simulink model "tb_mcu_closed_loop"  (R2026b)
values from neighbouring files (symbols this model uses):
  P = evalin('base', 'P')    [elec_harness.m]    (also in mcu_can1_roundtrip.m; mcu_can2_roundtrip.m; mcu_cl_input.m; mcu_ctrl_harness.m)
  Ts = prm(1)    [mcu_cl_track_dyn.m]    (also in mcu_ctrl_harness.m = evalin('base', tsExpr))
undefined symbols (not defined in the file or in its folder): DiscIntNeverNeededParam
libraries: simulink x57, robotmobilelib x1
(part 1 of 2)
settings Model: Creator=aomar  LastModifiedBy=aomar

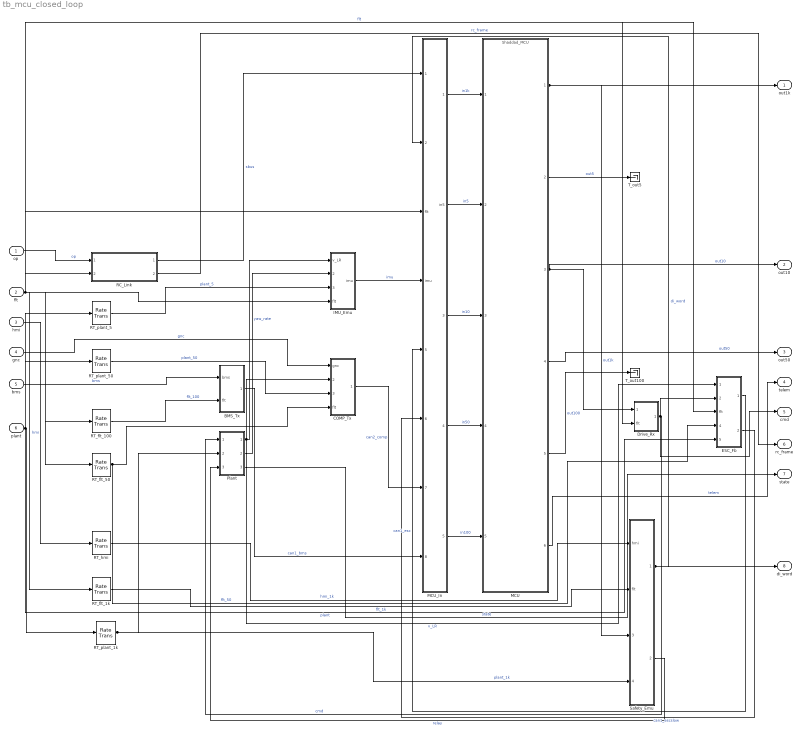
== system tb_mcu_closed_loop ==
  op : Inport  OutDataTypeStr=Bus: Bus_OperatorCmd  SampleTime=Ts.ctrl  BusOutputAsStruct=on
  flt : Inport  Port=2  OutDataTypeStr=Bus: Bus_FaultInject  SampleTime=Ts.ctrl  BusOutputAsStruct=on
  hmi : Inport  Port=3  OutDataTypeStr=Bus: Bus_HmiInputs  SampleTime=Ts.ctrl  BusOutputAsStruct=on
  gnc : Inport  Port=4  OutDataTypeStr=Bus: Bus_GncCmd  SampleTime=Ts.comm  BusOutputAsStruct=on
  bms : Inport  Port=5  OutDataTypeStr=Bus: Bus_BMS_Telemetry  SampleTime=Ts.hk  BusOutputAsStruct=on
  plant : Inport  Port=6  OutDataTypeStr=double  PortDimensions=9  SampleTime=Ts.ctrl
  BMS_Tx : Subsystem
  COMP_Tx : Subsystem
  Drive_Rx : Subsystem
  ESC_Fb : Subsystem
  IMU_Emu : Subsystem
  MCU : ModelReference  ModelNameDialog=Shaddad_MCU  SimulationMode=Normal  ModelReferenceVersion=1.1
  MCU_In : Subsystem
  Plant : Subsystem
  RC_Link : Subsystem  ReferencedSubsystem=RC_Link_Sim
  RT_flt_100 : RateTransition  InitialCondition=P.ic.Bus_FaultInject  OutPortSampleTime=Ts.hk
  RT_flt_1k : RateTransition  InitialCondition=P.ic.Bus_FaultInject  OutPortSampleTime=Ts.base
  RT_flt_50 : RateTransition  InitialCondition=P.ic.Bus_FaultInject  OutPortSampleTime=Ts.comm
  RT_hmi : RateTransition  InitialCondition=P.ic.Bus_HmiInputs  OutPortSampleTime=Ts.base
  RT_plant_1k : RateTransition  InitialCondition=[1 0 0 0 0 0 0 0 0]  OutPortSampleTime=Ts.base
  RT_plant_5 : RateTransition  InitialCondition=[1 0 0 0 0 0 0 0 0]  OutPortSampleTime=Ts.imu
  RT_plant_50 : RateTransition  InitialCondition=[1 0 0 0 0 0 0 0 0]  OutPortSampleTime=Ts.comm
  Safety_Emu : Subsystem
  T_out100 : Terminator
  T_out5 : Terminator
  out1k : Outport  OutDataTypeStr=Bus: Bus_McuOut1k
  out10 : Outport  Port=2  OutDataTypeStr=Bus: Bus_McuOut10
  out50 : Outport  Port=3  OutDataTypeStr=Bus: Bus_McuOut50
  telem : Outport  Port=4  OutDataTypeStr=Bus: Bus_FwTelemetry
  cmd : Outport  Port=5  OutDataTypeStr=Bus: Bus_DriveCmd
  rc_frame : Outport  Port=6  OutDataTypeStr=Bus: Bus_RcFrame
  state : Outport  Port=7  OutDataTypeStr=double
  di_word : Outport  Port=8  OutDataTypeStr=uint16
  wires:
  op/1 -> RC_Link/1  "op"
  hmi/1 -> RT_hmi/1  "hmi"
  gnc/1 -> COMP_Tx/1(gnc)  "gnc"
  bms/1 -> BMS_Tx/1(bms)  "bms"
  RT_plant_5/1 -> IMU_Emu/3(plant)  "plant_5"
  RT_plant_50/1 -> COMP_Tx/3(plant)  "plant_50"
  RT_flt_100/1 -> BMS_Tx/2(flt)  "flt_100"
  RT_flt_50/1 -> COMP_Tx/4(flt), ESC_Fb/4(flt_50)  "flt_50"
  RT_hmi/1 -> Safety_Emu/1(hmi)  "hmi_1k"
  RT_flt_1k/1 -> Safety_Emu/2(flt)  "flt_1k"
  RT_plant_1k/1 -> Plant/2(plant), Safety_Emu/4(plant)  "plant_1k"
  RC_Link/1 -> MCU_In/1(sbus)  "sbus"
  RC_Link/2 -> rc_frame/1  "rc_frame"
  BMS_Tx/1(frames) -> MCU_In/8(can1_bms)  "can1_bms"
  Plant/1(v_LR) -> IMU_Emu/1(v_LR), COMP_Tx/2(v_LR), ESC_Fb/1(v_LR)  "v_LR"
  Plant/2(yaw_rate) -> IMU_Emu/2(yaw_rate)  "yaw_rate"
  Plant/3(state) -> state/1  "state"
  IMU_Emu/1(imu) -> MCU_In/4(imu)  "imu"
  COMP_Tx/1(frame) -> MCU_In/7(can2_comp)  "can2_comp"
  MCU_In/1(in1k) -> MCU/1  "in1k"
  MCU_In/2(in5) -> MCU/2  "in5"
  MCU_In/3(in10) -> MCU/3  "in10"
  MCU_In/4(in50) -> MCU/4  "in50"
  MCU_In/5(in100) -> MCU/5  "in100"
  MCU/1 -> Safety_Emu/3(out1k), out1k/1  "out1k"
  MCU/2 -> T_out5/1  "out5"
  MCU/3 -> Drive_Rx/1(out10), out10/1  "out10"
  MCU/4 -> out50/1  "out50"
  MCU/5 -> T_out100/1  "out100"
  MCU/6 -> telem/1  "telem"
  Safety_Emu/1(di_word) -> MCU_In/2(di_word), di_word/1  "di_word"
  Safety_Emu/2(relay) -> Plant/3(relay)  "relay"
  Drive_Rx/1(cmd) -> Plant/1(cmd), ESC_Fb/2(cmd), cmd/1  "cmd"
  ESC_Fb/1(esc_fast) -> MCU_In/5(can1_esc)  "can1_esc"
  ESC_Fb/2(esc_slow) -> MCU_In/6(can1_escslow)  "can1_escslow"
  flt/1 -> RT_flt_1k/1, RT_flt_50/1, Drive_Rx/2(flt), RT_flt_100/1, ESC_Fb/3(flt), MCU_In/3(flt), RC_Link/2, IMU_Emu/4(flt)  "flt"
  plant/1 -> RT_plant_1k/1, RT_plant_5/1, RT_plant_50/1, ESC_Fb/5(plant)  "plant"

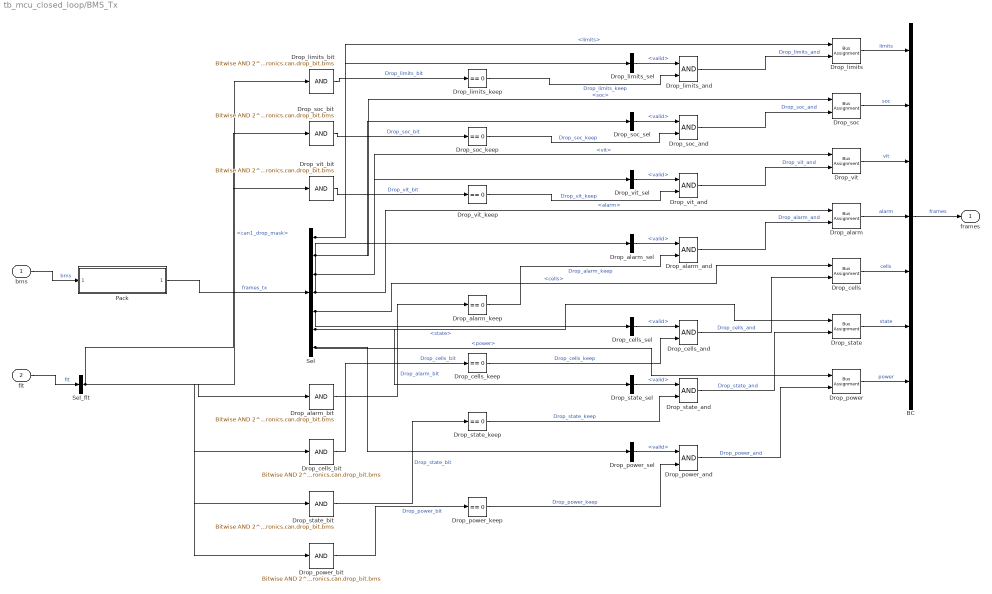
== system tb_mcu_closed_loop/BMS_Tx ==
  bms : Inport
  flt : Inport  Port=2
  BC : BusCreator  Inputs=7  OutDataTypeStr=Bus: Bus_Can1_Bms  NonVirtualBus=on
      settings: InheritFromInputs=off
  Drop_alarm : BusAssignment  AssignedSignals=valid
  Drop_alarm_and : Logic  AllPortsSameDT=off  OutDataTypeStr=boolean
  Drop_alarm_bit : simulink/Logic and Bit Operations/Bitwise Operator  logicop=AND  UseBitMask=on  BitMask=2^P.electronics.can.drop_bit.bms  BitMaskRealWorld=Stored Integer
  Drop_alarm_keep : simulink/Logic and Bit Operations/Compare To Zero  relop===  OutDataTypeStr=boolean
  Drop_alarm_sel : BusSelector  OutputSignals=valid
  Drop_cells : BusAssignment  AssignedSignals=valid
  Drop_cells_and : Logic  AllPortsSameDT=off  OutDataTypeStr=boolean
  Drop_cells_bit : simulink/Logic and Bit Operations/Bitwise Operator  logicop=AND  UseBitMask=on  BitMask=2^P.electronics.can.drop_bit.bms  BitMaskRealWorld=Stored Integer
  Drop_cells_keep : simulink/Logic and Bit Operations/Compare To Zero  relop===  OutDataTypeStr=boolean
  Drop_cells_sel : BusSelector  OutputSignals=valid
  Drop_limits : BusAssignment  AssignedSignals=valid
  Drop_limits_and : Logic  AllPortsSameDT=off  OutDataTypeStr=boolean
  Drop_limits_bit : simulink/Logic and Bit Operations/Bitwise Operator  logicop=AND  UseBitMask=on  BitMask=2^P.electronics.can.drop_bit.bms  BitMaskRealWorld=Stored Integer
  Drop_limits_keep : simulink/Logic and Bit Operations/Compare To Zero  relop===  OutDataTypeStr=boolean
  Drop_limits_sel : BusSelector  OutputSignals=valid
  Drop_power : BusAssignment  AssignedSignals=valid
  Drop_power_and : Logic  AllPortsSameDT=off  OutDataTypeStr=boolean
  Drop_power_bit : simulink/Logic and Bit Operations/Bitwise Operator  logicop=AND  UseBitMask=on  BitMask=2^P.electronics.can.drop_bit.bms  BitMaskRealWorld=Stored Integer
  Drop_power_keep : simulink/Logic and Bit Operations/Compare To Zero  relop===  OutDataTypeStr=boolean
  Drop_power_sel : BusSelector  OutputSignals=valid
  Drop_soc : BusAssignment  AssignedSignals=valid
  Drop_soc_and : Logic  AllPortsSameDT=off  OutDataTypeStr=boolean
  Drop_soc_bit : simulink/Logic and Bit Operations/Bitwise Operator  logicop=AND  UseBitMask=on  BitMask=2^P.electronics.can.drop_bit.bms  BitMaskRealWorld=Stored Integer
  Drop_soc_keep : simulink/Logic and Bit Operations/Compare To Zero  relop===  OutDataTypeStr=boolean
  Drop_soc_sel : BusSelector  OutputSignals=valid
  Drop_state : BusAssignment  AssignedSignals=valid
  Drop_state_and : Logic  AllPortsSameDT=off  OutDataTypeStr=boolean
  Drop_state_bit : simulink/Logic and Bit Operations/Bitwise Operator  logicop=AND  UseBitMask=on  BitMask=2^P.electronics.can.drop_bit.bms  BitMaskRealWorld=Stored Integer
  Drop_state_keep : simulink/Logic and Bit Operations/Compare To Zero  relop===  OutDataTypeStr=boolean
  Drop_state_sel : BusSelector  OutputSignals=valid
  Drop_vit : BusAssignment  AssignedSignals=valid
  Drop_vit_and : Logic  AllPortsSameDT=off  OutDataTypeStr=boolean
  Drop_vit_bit : simulink/Logic and Bit Operations/Bitwise Operator  logicop=AND  UseBitMask=on  BitMask=2^P.electronics.can.drop_bit.bms  BitMaskRealWorld=Stored Integer
  Drop_vit_keep : simulink/Logic and Bit Operations/Compare To Zero  relop===  OutDataTypeStr=boolean
  Drop_vit_sel : BusSelector  OutputSignals=valid
  Pack : Subsystem  ReferencedSubsystem=bms_can_pack
  Sel : BusSelector  OutputSignals=limits,soc,vit,alarm,cells,state,power
  Sel_flt : BusSelector  OutputSignals=can1_drop_mask
  frames : Outport
  wires:
  bms/1 -> Pack/1  "bms"
  flt/1 -> Sel_flt/1  "flt"
  Sel_flt/1 -> Drop_limits_bit/1, Drop_soc_bit/1, Drop_vit_bit/1, Drop_power_bit/1, Drop_state_bit/1, Drop_cells_bit/1, Drop_alarm_bit/1  "<can1_drop_mask>"
  Pack/1 -> Sel/1  "frames_tx"
  Sel/1 -> Drop_limits/1, Drop_limits_sel/1  "<limits>"
  Sel/2 -> Drop_soc/1, Drop_soc_sel/1  "<soc>"
  Sel/3 -> Drop_vit/1, Drop_vit_sel/1  "<vit>"
  Sel/4 -> Drop_alarm/1, Drop_alarm_sel/1  "<alarm>"
  Sel/5 -> Drop_cells/1, Drop_cells_sel/1  "<cells>"
  Sel/6 -> Drop_state_sel/1, Drop_state/1  "<state>"
  Sel/7 -> Drop_power_sel/1, Drop_power/1  "<power>"
  Drop_limits_bit/1 -> Drop_limits_keep/1  "Drop_limits_bit"
  Drop_soc_bit/1 -> Drop_soc_keep/1  "Drop_soc_bit"
  Drop_vit_bit/1 -> Drop_vit_keep/1  "Drop_vit_bit"
  Drop_alarm_bit/1 -> Drop_alarm_keep/1  "Drop_alarm_bit"
  Drop_cells_bit/1 -> Drop_cells_keep/1  "Drop_cells_bit"
  Drop_state_bit/1 -> Drop_state_keep/1  "Drop_state_bit"
  Drop_power_bit/1 -> Drop_power_keep/1  "Drop_power_bit"
  Drop_limits_keep/1 -> Drop_limits_and/2  "Drop_limits_keep"
  Drop_soc_keep/1 -> Drop_soc_and/2  "Drop_soc_keep"
  Drop_vit_keep/1 -> Drop_vit_and/2  "Drop_vit_keep"
  Drop_alarm_keep/1 -> Drop_alarm_and/2  "Drop_alarm_keep"
  Drop_cells_keep/1 -> Drop_cells_and/2  "Drop_cells_keep"
  Drop_state_keep/1 -> Drop_state_and/2  "Drop_state_keep"
  Drop_power_keep/1 -> Drop_power_and/2  "Drop_power_keep"
  Drop_limits_sel/1 -> Drop_limits_and/1  "<valid>"
  Drop_soc_sel/1 -> Drop_soc_and/1  "<valid>"
  Drop_vit_sel/1 -> Drop_vit_and/1  "<valid>"
  Drop_alarm_sel/1 -> Drop_alarm_and/1  "<valid>"
  Drop_cells_sel/1 -> Drop_cells_and/1  "<valid>"
  Drop_state_sel/1 -> Drop_state_and/1  "<valid>"
  Drop_power_sel/1 -> Drop_power_and/1  "<valid>"
  Drop_limits_and/1 -> Drop_limits/2  "Drop_limits_and"
  Drop_soc_and/1 -> Drop_soc/2  "Drop_soc_and"
  Drop_vit_and/1 -> Drop_vit/2  "Drop_vit_and"
  Drop_alarm_and/1 -> Drop_alarm/2  "Drop_alarm_and"
  Drop_cells_and/1 -> Drop_cells/2  "Drop_cells_and"
  Drop_state_and/1 -> Drop_state/2  "Drop_state_and"
  Drop_power_and/1 -> Drop_power/2  "Drop_power_and"
  Drop_limits/1 -> BC/1  "limits"
  Drop_soc/1 -> BC/2  "soc"
  Drop_vit/1 -> BC/3  "vit"
  Drop_alarm/1 -> BC/4  "alarm"
  Drop_cells/1 -> BC/5  "cells"
  Drop_state/1 -> BC/6  "state"
  Drop_power/1 -> BC/7  "power"
  BC/1 -> frames/1  "frames"

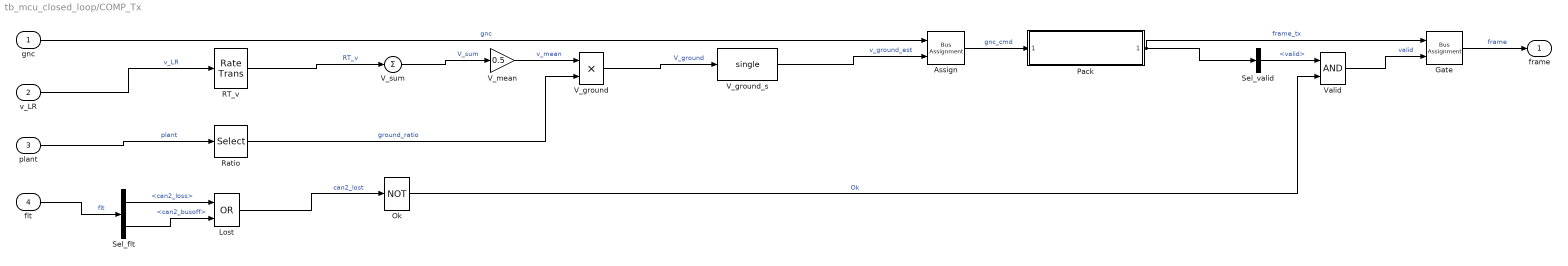
== system tb_mcu_closed_loop/COMP_Tx ==
  gnc : Inport
  v_LR : Inport  Port=2
  plant : Inport  Port=3
  flt : Inport  Port=4
  Assign : BusAssignment  AssignedSignals=v_ground_est
  Gate : BusAssignment  AssignedSignals=valid
  Lost : Logic  Operator=OR  AllPortsSameDT=off  OutDataTypeStr=boolean
  Ok : Logic  Operator=NOT  Inputs=1  AllPortsSameDT=off  OutDataTypeStr=boolean
  Pack : Subsystem  ReferencedSubsystem=can2_comp_cmd_pack
  RT_v : RateTransition  InitialCondition=[0 0]  OutPortSampleTime=Ts.comm
  Ratio : Selector  InputPortWidth=9  IndexOptions=Index vector (dialog)  Indices=4  OutputSizes=1
  Sel_flt : BusSelector  OutputSignals=can2_loss,can2_busoff
  Sel_valid : BusSelector  OutputSignals=valid
  V_ground : Product  Inputs=**
  V_ground_s : DataTypeConversion  OutDataTypeStr=single  RndMeth=Round
  V_mean : Gain  Gain=0.5
  V_sum : Sum  Inputs=+
  Valid : Logic  AllPortsSameDT=off  OutDataTypeStr=boolean
  frame : Outport
  wires:
  gnc/1 -> Assign/1  "gnc"
  v_LR/1 -> RT_v/1  "v_LR"
  plant/1 -> Ratio/1  "plant"
  flt/1 -> Sel_flt/1  "flt"
  Sel_flt/1 -> Lost/1  "<can2_loss>"
  Sel_flt/2 -> Lost/2  "<can2_busoff>"
  Lost/1 -> Ok/1  "can2_lost"
  RT_v/1 -> V_sum/1  "RT_v"
  Ratio/1 -> V_ground/2  "ground_ratio"
  V_sum/1 -> V_mean/1  "V_sum"
  Ok/1 -> Valid/2  "Ok"
  V_mean/1 -> V_ground/1  "v_mean"
  V_ground/1 -> V_ground_s/1  "V_ground"
  V_ground_s/1 -> Assign/2  "v_ground_est"
  Assign/1 -> Pack/1  "gnc_cmd"
  Pack/1 -> Sel_valid/1, Gate/1  "frame_tx"
  Sel_valid/1 -> Valid/1  "<valid>"
  Valid/1 -> Gate/2  "valid"
  Gate/1 -> frame/1  "frame"

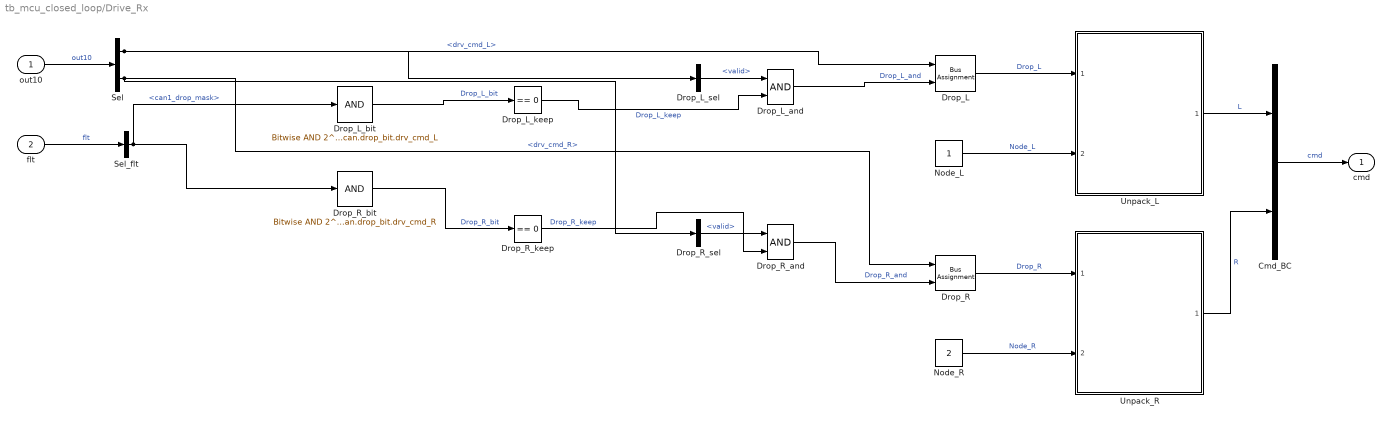
== system tb_mcu_closed_loop/Drive_Rx ==
  out10 : Inport
  flt : Inport  Port=2
  Cmd_BC : BusCreator  Inputs=2  OutDataTypeStr=Bus: Bus_DriveCmd  NonVirtualBus=on
      settings: InheritFromInputs=off
  Drop_L : BusAssignment  AssignedSignals=valid
  Drop_L_and : Logic  AllPortsSameDT=off  OutDataTypeStr=boolean
  Drop_L_bit : simulink/Logic and Bit Operations/Bitwise Operator  logicop=AND  UseBitMask=on  BitMask=2^P.electronics.can.drop_bit.drv_cmd_L  BitMaskRealWorld=Stored Integer
  Drop_L_keep : simulink/Logic and Bit Operations/Compare To Zero  relop===  OutDataTypeStr=boolean
  Drop_L_sel : BusSelector  OutputSignals=valid
  Drop_R : BusAssignment  AssignedSignals=valid
  Drop_R_and : Logic  AllPortsSameDT=off  OutDataTypeStr=boolean
  Drop_R_bit : simulink/Logic and Bit Operations/Bitwise Operator  logicop=AND  UseBitMask=on  BitMask=2^P.electronics.can.drop_bit.drv_cmd_R  BitMaskRealWorld=Stored Integer
  Drop_R_keep : simulink/Logic and Bit Operations/Compare To Zero  relop===  OutDataTypeStr=boolean
  Drop_R_sel : BusSelector  OutputSignals=valid
  Node_L : Constant  OutDataTypeStr=uint8  SampleTime=Ts.ctrl
  Node_R : Constant  Value=2  OutDataTypeStr=uint8  SampleTime=Ts.ctrl
  Sel : BusSelector  OutputSignals=can1_drv.drv_cmd_L,can1_drv.drv_cmd_R
  Sel_flt : BusSelector  OutputSignals=can1_drop_mask
  Unpack_L : Subsystem  ReferencedSubsystem=drive_cmd_unpack
  Unpack_R : Subsystem  ReferencedSubsystem=drive_cmd_unpack
  cmd : Outport
  wires:
  out10/1 -> Sel/1  "out10"
  flt/1 -> Sel_flt/1  "flt"
  Sel/1 -> Drop_L_sel/1, Drop_L/1  "<drv_cmd_L>"
  Sel/2 -> Drop_R/1, Drop_R_sel/1  "<drv_cmd_R>"
  Sel_flt/1 -> Drop_R_bit/1, Drop_L_bit/1  "<can1_drop_mask>"
  Drop_L_bit/1 -> Drop_L_keep/1  "Drop_L_bit"
  Drop_R_bit/1 -> Drop_R_keep/1  "Drop_R_bit"
  Drop_L_keep/1 -> Drop_L_and/2  "Drop_L_keep"
  Drop_R_keep/1 -> Drop_R_and/2  "Drop_R_keep"
  Drop_L_sel/1 -> Drop_L_and/1  "<valid>"
  Drop_R_sel/1 -> Drop_R_and/1  "<valid>"
  Drop_L_and/1 -> Drop_L/2  "Drop_L_and"
  Drop_R_and/1 -> Drop_R/2  "Drop_R_and"
  Node_L/1 -> Unpack_L/2  "Node_L"
  Node_R/1 -> Unpack_R/2  "Node_R"
  Drop_L/1 -> Unpack_L/1  "Drop_L"
  Drop_R/1 -> Unpack_R/1  "Drop_R"
  Unpack_L/1 -> Cmd_BC/1  "L"
  Unpack_R/1 -> Cmd_BC/2  "R"
  Cmd_BC/1 -> cmd/1  "cmd"

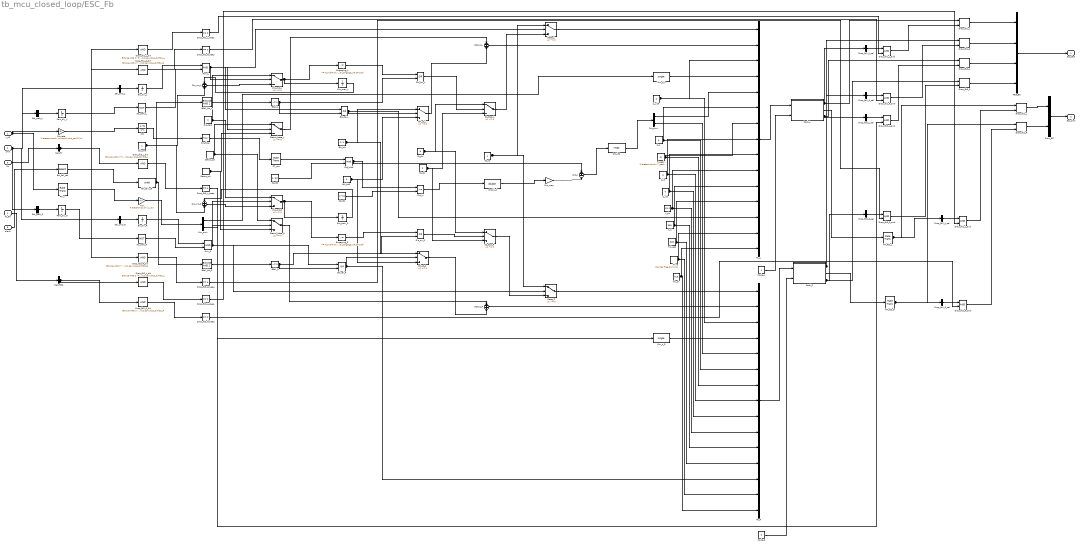
== system tb_mcu_closed_loop/ESC_Fb ==
  v_LR : Inport
  cmd : Inport  Port=2
  flt : Inport  Port=3
  flt_50 : Inport  Port=4
  plant : Inport  Port=5
  Alive : simulink/Sources/Counter Free-Running  NumBits=8  tsamp=Ts.ctrl
  Bfail_L : simulink/Logic and Bit Operations/Compare To Zero  relop=~=  OutDataTypeStr=boolean
  Bfail_R : simulink/Logic and Bit Operations/Compare To Zero  relop=~=  OutDataTypeStr=boolean
  Bfail_bit_L : simulink/Logic and Bit Operations/Bitwise Operator  logicop=AND  UseBitMask=on  BitMask=1  BitMaskRealWorld=Stored Integer
  Bfail_bit_R : simulink/Logic and Bit Operations/Bitwise Operator  logicop=AND  UseBitMask=on  BitMask=2  BitMaskRealWorld=Stored Integer
  Brk_bit : Constant  Value=2^4  OutDataTypeStr=uint16  SampleTime=Ts.ctrl
  Brk_bit0 : Constant  Value=0  OutDataTypeStr=uint16  SampleTime=Ts.ctrl
  Brk_fail_sel : Selector  InputPortWidth=9  IndexOptions=Index vector (dialog)  Indices=6  OutputSizes=1
  Brk_fail_u8 : DataTypeConversion  OutDataTypeStr=uint8  RndMeth=Round
  Brk_rel_L : Logic  Operator=OR  AllPortsSameDT=off  OutDataTypeStr=boolean
  Brk_rel_R : Logic  Operator=OR  AllPortsSameDT=off  OutDataTypeStr=boolean
  Brk_st_L : Switch  Criteria=u2 ~= 0  SaturateOnIntegerOverflow=off  InputSameDT=off
  Brk_st_R : Switch  Criteria=u2 ~= 0  SaturateOnIntegerOverflow=off  InputSameDT=off
  C2p31 : Constant  Value=2^31  OutDataTypeStr=double  SampleTime=Ts.ctrl
  C2p32 : Constant  Value=2^32  OutDataTypeStr=double  SampleTime=Ts.ctrl
  Cnt : DiscreteIntegrator  InitialCondition=[0 0]  SampleTime=Ts.base  ICPrevOutput=DiscIntNeverNeededParam  ICPrevScaledInput=DiscIntNeverNeededParam
  Cnt_dmx : Demux  Outputs=2
  Cnt_floor : Rounding
  Cnt_hi : RelationalOperator  OutDataTypeStr=boolean  RndMeth=Simplest  InputSameDT=off
  Cnt_hi_d : DataTypeConversion  OutDataTypeStr=double  RndMeth=Round
  Cnt_i32 : DataTypeConversion  OutDataTypeStr=int32  RndMeth=Round
  Cnt_mod : Math  Operator=mod
  Cnt_rate : Gain  Gain=P.electronics.drv.k_v2w*P.electronics.drv.enc_cpr/(2*pi)
  Cnt_s : Sum  Inputs=+-
  Cnt_wrap : Gain  Gain=2^32
  Dis_cnt_L : Switch  Criteria=u2 ~= 0  SaturateOnIntegerOverflow=off  InputSameDT=off
  Dis_cnt_R : Switch  Criteria=u2 ~= 0  SaturateOnIntegerOverflow=off  InputSameDT=off
  Dis_inc_L : Sum  OutDataTypeStr=uint16  SaturateOnIntegerOverflow=on
  Dis_inc_R : Sum  OutDataTypeStr=uint16  SaturateOnIntegerOverflow=on
  Dis_on_L : Logic  Operator=OR  AllPortsSameDT=off  OutDataTypeStr=boolean
  Dis_on_R : Logic  Operator=OR  AllPortsSameDT=off  OutDataTypeStr=boolean
  Dis_one : Constant  OutDataTypeStr=uint16  SampleTime=Ts.ctrl
  Dis_prev_L : UnitDelay  InitialCondition=1000  SampleTime=Ts.ctrl
  Dis_prev_R : UnitDelay  InitialCondition=1000  SampleTime=Ts.ctrl
  Dis_zero : Constant  Value=0  OutDataTypeStr=uint16  SampleTime=Ts.ctrl
  Drop_fb1_L : BusAssignment  AssignedSignals=valid
  Drop_fb1_L_and : Logic  AllPortsSameDT=off  OutDataTypeStr=boolean
  Drop_fb1_L_bit : simulink/Logic and Bit Operations/Bitwise Operator  logicop=AND  UseBitMask=on  BitMask=2^P.electronics.can.drop_bit.fb1_L  BitMaskRealWorld=Stored Integer
  Drop_fb1_L_keep : simulink/Logic and Bit Operations/Compare To Zero  relop===  OutDataTypeStr=boolean
  Drop_fb1_L_sel : BusSelector  OutputSignals=valid
  Drop_fb1_R : BusAssignment  AssignedSignals=valid
  Drop_fb1_R_and : Logic  AllPortsSameDT=off  OutDataTypeStr=boolean
  Drop_fb1_R_bit : simulink/Logic and Bit Operations/Bitwise Operator  logicop=AND  UseBitMask=on  BitMask=2^P.electronics.can.drop_bit.fb1_R  BitMaskRealWorld=Stored Integer
  Drop_fb1_R_keep : simulink/Logic and Bit Operations/Compare To Zero  relop===  OutDataTypeStr=boolean
  Drop_fb1_R_sel : BusSelector  OutputSignals=valid
  Drop_fb2_L : BusAssignment  AssignedSignals=valid
  Drop_fb2_L_and : Logic  AllPortsSameDT=off  OutDataTypeStr=boolean
  Drop_fb2_L_bit : simulink/Logic and Bit Operations/Bitwise Operator  logicop=AND  UseBitMask=on  BitMask=2^P.electronics.can.drop_bit.fb2_L  BitMaskRealWorld=Stored Integer
  Drop_fb2_L_keep : simulink/Logic and Bit Operations/Compare To Zero  relop===  OutDataTypeStr=boolean
  Drop_fb2_L_sel : BusSelector  OutputSignals=valid
  Drop_fb2_R : BusAssignment  AssignedSignals=valid
  Drop_fb2_R_and : Logic  AllPortsSameDT=off  OutDataTypeStr=boolean
  Drop_fb2_R_bit : simulink/Logic and Bit Operations/Bitwise Operator  logicop=AND  UseBitMask=on  BitMask=2^P.electronics.can.drop_bit.fb2_R  BitMaskRealWorld=Stored Integer
  Drop_fb2_R_keep : simulink/Logic and Bit Operations/Compare To Zero  relop===  OutDataTypeStr=boolean
  Drop_fb2_R_sel : BusSelector  OutputSignals=valid
  Drop_fb3_L : BusAssignment  AssignedSignals=valid
  Drop_fb3_L_and : Logic  AllPortsSameDT=off  OutDataTypeStr=boolean
  Drop_fb3_L_bit : simulink/Logic and Bit Operations/Bitwise Operator  logicop=AND  UseBitMask=on  BitMask=2^P.electronics.can.drop_bit.fb3_L  BitMaskRealWorld=Stored Integer
  Drop_fb3_L_keep : simulink/Logic and Bit Operations/Compare To Zero  relop===  OutDataTypeStr=boolean
  Drop_fb3_L_sel : BusSelector  OutputSignals=valid
  Drop_fb3_R : BusAssignment  AssignedSignals=valid
  Drop_fb3_R_and : Logic  AllPortsSameDT=off  OutDataTypeStr=boolean
  Drop_fb3_R_bit : simulink/Logic and Bit Operations/Bitwise Operator  logicop=AND  UseBitMask=on  BitMask=2^P.electronics.can.drop_bit.fb3_R  BitMaskRealWorld=Stored Integer
  Drop_fb3_R_keep : simulink/Logic and Bit Operations/Compare To Zero  relop===  OutDataTypeStr=boolean
  Drop_fb3_R_sel : BusSelector  OutputSignals=valid
  En_dly_L : UnitDelay  InitialCondition=false  SampleTime=-1
  En_dly_R : UnitDelay  InitialCondition=false  SampleTime=-1
  Engaging_L : simulink/Logic and Bit Operations/Compare To Constant  relop=<=  const=round(P.drive.brake.t_engage_wait/Ts.ctrl)  OutDataTypeStr=boolean
  Engaging_R : simulink/Logic and Bit Operations/Compare To Constant  relop=<=  const=round(P.drive.brake.t_engage_wait/Ts.ctrl)  OutDataTypeStr=boolean
  Fast_BC : BusCreator  Inputs=4  OutDataTypeStr=Bus: Bus_Can1_EscFast  NonVirtualBus=on
      settings: InheritFromInputs=off
  Fb_L : BusCreator  Inputs=15  OutDataTypeStr=Bus: Bus_DriveSideFb  NonVirtualBus=on
      settings: InheritFromInputs=off
  Fb_R : BusCreator  Inputs=15  OutDataTypeStr=Bus: Bus_DriveSideFb  NonVirtualBus=on
      settings: InheritFromInputs=off
  No_park_L : Logic  Operator=NOT  Inputs=1  AllPortsSameDT=off  OutDataTypeStr=boolean
  No_park_R : Logic  Operator=NOT  Inputs=1  AllPortsSameDT=off  OutDataTypeStr=boolean
  Node_L : Constant  OutDataTypeStr=uint8  SampleTime=Ts.ctrl
  Node_R : Constant  Value=2  OutDataTypeStr=uint8  SampleTime=Ts.ctrl
  Pack_L : Subsystem  ReferencedSubsystem=drive_fb_pack
  Pack_R : Subsystem  ReferencedSubsystem=drive_fb_pack
  Park_dly_L : UnitDelay  InitialCondition=true  SampleTime=-1
  Park_dly_R : UnitDelay  InitialCondition=true  SampleTime=-1
  RT_cnt : RateTransition  InitialCondition=[0 0]  OutPortSampleTime=Ts.ctrl
  RT_fb2_L : RateTransition  InitialCondition=P.ic.Bus_CanFrame8  OutPortSampleTime=Ts.comm
  RT_fb2_R : RateTransition  InitialCondition=P.ic.Bus_CanFrame8  OutPortSampleTime=Ts.comm
  RT_v : RateTransition  InitialCondition=[0 0]  OutPortSampleTime=Ts.ctrl
  Run_L : Logic  AllPortsSameDT=off  OutDataTypeStr=boolean
  Run_R : Logic  AllPortsSameDT=off  OutDataTypeStr=boolean
  Rx_ok : Constant  Value=true  OutDataTypeStr=boolean  SampleTime=Ts.ctrl
  Sel_cmd_L : BusSelector  OutputSignals=L.enable
  Sel_cmd_R : BusSelector  OutputSignals=R.enable
  Sel_flt : BusSelector  OutputSignals=can1_drop_mask
  Sel_flt50 : BusSelector  OutputSignals=can1_drop_mask
  Sel_park_L : BusSelector  OutputSignals=L.park_req
  Sel_park_R : BusSelector  OutputSignals=R.park_req
  Slow_BC : BusCreator  Inputs=2  OutDataTypeStr=Bus: Bus_Can1_EscSlow  NonVirtualBus=on
      settings: InheritFromInputs=off
  St_dis : Constant  Value=5  OutDataTypeStr=uint8  SampleTime=Ts.ctrl
  St_op : Constant  Value=4  OutDataTypeStr=uint8  SampleTime=Ts.ctrl
  St_rdy : Constant  Value=2  OutDataTypeStr=uint8  SampleTime=Ts.ctrl
  St_stop_L : Switch  Criteria=u2 ~= 0  SaturateOnIntegerOverflow=off  InputSameDT=off
  St_stop_R : Switch  Criteria=u2 ~= 0  SaturateOnIntegerOverflow=off  InputSameDT=off
  State_L : Switch  Criteria=u2 ~= 0  SaturateOnIntegerOverflow=off  InputSameDT=off
  State_R : Switch  Criteria=u2 ~= 0  SaturateOnIntegerOverflow=off  InputSameDT=off
  Status_L : Sum  OutDataTypeStr=uint16
  Status_R : Sum  OutDataTypeStr=uint16
  Status_base_L : Switch  Criteria=u2 ~= 0  SaturateOnIntegerOverflow=off  InputSameDT=off
  Status_base_R : Switch  Criteria=u2 ~= 0  SaturateOnIntegerOverflow=off  InputSameDT=off
  Status_op : Constant  Value=2^0 + 2^1 + 2^5  OutDataTypeStr=uint16  SampleTime=Ts.ctrl
  Status_rdy : Constant  Value=2^0 + 2^5  OutDataTypeStr=uint16  SampleTime=Ts.ctrl
  T_K : Constant  Value=300  OutDataTypeStr=single  SampleTime=Ts.ctrl
  T_K_esc : Constant  Value=300  OutDataTypeStr=single  SampleTime=Ts.ctrl
  T_peak : Constant  Value=P.electronics.drv.T_peak  OutDataTypeStr=single  SampleTime=Ts.ctrl
  V_dc : Constant  Value=51.2  OutDataTypeStr=single  SampleTime=Ts.ctrl
  Wm : Gain  Gain=P.electronics.drv.k_v2w
  Wm_dmx : Demux  Outputs=2
  Wm_s_L : DataTypeConversion  OutDataTypeStr=single  RndMeth=Round
  Wm_s_R : DataTypeConversion  OutDataTypeStr=single  RndMeth=Round
  Z_idc : Constant  Value=0  OutDataTypeStr=single  SampleTime=Ts.ctrl
  Z_iq : Constant  Value=0  OutDataTypeStr=single  SampleTime=Ts.ctrl
  Z_s : Constant  Value=0  OutDataTypeStr=single  SampleTime=Ts.ctrl
  Z_u16 : Constant  Value=0  OutDataTypeStr=uint16  SampleTime=Ts.ctrl
  esc_fast : Outport
  esc_slow : Outport  Port=2
  wires:
  v_LR/1 -> RT_v/1, Cnt_rate/1  "v_LR"
  cmd/1 -> Sel_cmd_R/1, Sel_park_R/1, Sel_cmd_L/1, Sel_park_L/1  "cmd"
  flt/1 -> Sel_flt/1  "flt"
  flt_50/1 -> Sel_flt50/1  "flt_50"
  plant/1 -> Brk_fail_sel/1  "plant"
  Sel_park_L/1 -> Park_dly_L/1  "<park_req>"
  Sel_park_R/1 -> Park_dly_R/1  "<park_req>"
  Sel_flt/1 -> Drop_fb3_R_bit/1, Drop_fb1_L_bit/1, Drop_fb1_R_bit/1, Drop_fb3_L_bit/1  "<can1_drop_mask>"
  Sel_flt50/1 -> Drop_fb2_R_bit/1, Drop_fb2_L_bit/1  "<can1_drop_mask>"
  Cnt_rate/1 -> Cnt/1  "count_rate"
  Park_dly_L/1 -> No_park_L/1  "park_req_L"
  Park_dly_R/1 -> No_park_R/1  "park_req_R"
  Brk_fail_sel/1 -> Brk_fail_u8/1  "brake_fail_d"
  RT_v/1 -> Wm/1  "RT_v"
  Sel_cmd_L/1 -> En_dly_L/1  "<enable>"
  Sel_cmd_R/1 -> En_dly_R/1  "<enable>"
  No_park_L/1 -> Run_L/2  "No_park_L"
  Dis_one/1 -> Dis_inc_R/2, Dis_inc_L/2  "Dis_one"
  Wm/1 -> Wm_dmx/1  "w_m"
  No_park_R/1 -> Run_R/2  "No_park_R"
  En_dly_L/1 -> Run_L/1  "enable_L"
  Cnt/1 -> Cnt_floor/1  "counts"
  En_dly_R/1 -> Run_R/1  "enable_R"
  Drop_fb1_L_bit/1 -> Drop_fb1_L_keep/1  "Drop_fb1_L_bit"
  Drop_fb1_R_bit/1 -> Drop_fb1_R_keep/1  "Drop_fb1_R_bit"
  Drop_fb3_L_bit/1 -> Drop_fb3_L_keep/1  "Drop_fb3_L_bit"
  Drop_fb3_R_bit/1 -> Drop_fb3_R_keep/1  "Drop_fb3_R_bit"
  Drop_fb2_L_bit/1 -> Drop_fb2_L_keep/1  "Drop_fb2_L_bit"
  Drop_fb2_R_bit/1 -> Drop_fb2_R_keep/1  "Drop_fb2_R_bit"
  Brk_fail_u8/1 -> Bfail_bit_R/1, Bfail_bit_L/1  "brake_fail"
  Wm_dmx/1 -> Wm_s_L/1  "Wm_dmx_1"
  Wm_dmx/2 -> Wm_s_R/1  "Wm_dmx_2"
  Dis_inc_L/1 -> Dis_cnt_L/3  "Dis_inc_L"
  Dis_inc_R/1 -> Dis_cnt_R/3  "Dis_inc_R"
  Drop_fb1_L_keep/1 -> Drop_fb1_L_and/2  "Drop_fb1_L_keep"
  Drop_fb1_R_keep/1 -> Drop_fb1_R_and/2  "Drop_fb1_R_keep"
  Run_L/1 -> Status_base_L/2, Brk_rel_L/1, State_L/2, Dis_cnt_L/2  "run_L"
  Cnt_floor/1 -> RT_cnt/1  "Cnt_floor"
  Status_rdy/1 -> Status_base_R/3, Status_base_L/3  "Status_rdy"
  Drop_fb3_L_keep/1 -> Drop_fb3_L_and/2  "Drop_fb3_L_keep"
  Drop_fb3_R_keep/1 -> Drop_fb3_R_and/2  "Drop_fb3_R_keep"
  Drop_fb2_L_keep/1 -> Drop_fb2_L_and/2  "Drop_fb2_L_keep"
  Drop_fb2_R_keep/1 -> Drop_fb2_R_and/2  "Drop_fb2_R_keep"
  Bfail_bit_L/1 -> Bfail_L/1  "Bfail_bit_L"
  Dis_zero/1 -> Dis_cnt_R/1, Dis_cnt_L/1  "Dis_zero"
  Run_R/1 -> State_R/2, Dis_cnt_R/2, Status_base_R/2, Brk_rel_R/1  "run_R"
  Bfail_bit_R/1 -> Bfail_R/1  "Bfail_bit_R"
  Status_op/1 -> Status_base_R/1, Status_base_L/1  "Status_op"
  Bfail_L/1 -> Dis_on_L/2, Brk_rel_L/2  "brake_fail_L"
  C2p32/1 -> Cnt_mod/2  "C2p32"
  Bfail_R/1 -> Dis_on_R/2, Brk_rel_R/2  "brake_fail_R"
  RT_cnt/1 -> Cnt_mod/1  "RT_cnt"
  Dis_cnt_L/1 -> Engaging_L/1, Dis_prev_L/1  "dis_cnt_L"
  Status_base_L/1 -> Status_L/1  "status_base_L"
  Dis_cnt_R/1 -> Engaging_R/1, Dis_prev_R/1  "dis_cnt_R"
  Status_base_R/1 -> Status_R/1  "status_base_R"
  Engaging_L/1 -> Dis_on_L/1  "engaging_L"
  Brk_bit/1 -> Brk_st_R/1, Brk_st_L/1  "Brk_bit"
  C2p31/1 -> Cnt_hi/2  "C2p31"
  Engaging_R/1 -> Dis_on_R/1  "engaging_R"
  Brk_rel_R/1 -> Fb_R/13, Brk_st_R/2  "brake_released_R"
  Dis_prev_L/1 -> Dis_inc_L/1  "dis_prev_L"
  Dis_prev_R/1 -> Dis_inc_R/1  "dis_prev_R"
  Brk_rel_L/1 -> Fb_L/13, Brk_st_L/2  "brake_released_L"
  Brk_bit0/1 -> Brk_st_R/3, Brk_st_L/3  "Brk_bit0"
  Cnt_mod/1 -> Cnt_hi/1, Cnt_s/1  "Cnt_mod"
  Dis_on_L/1 -> St_stop_L/2  "Dis_on_L"
  St_dis/1 -> St_stop_R/1, St_stop_L/1  "St_dis"
  Cnt_hi/1 -> Cnt_hi_d/1  "Cnt_hi"
  Dis_on_R/1 -> St_stop_R/2  "Dis_on_R"
  St_rdy/1 -> St_stop_R/3, St_stop_L/3  "St_rdy"
  Brk_st_L/1 -> Status_L/2  "Brk_st_L"
  Brk_st_R/1 -> Status_R/2  "Brk_st_R"
  Status_L/1 -> Fb_L/2  "status"
  Status_R/1 -> Fb_R/2  "status"
  St_op/1 -> State_L/1, State_R/1  "St_op"
  St_stop_L/1 -> State_L/3  "St_stop_L"
  St_stop_R/1 -> State_R/3  "St_stop_R"
  Cnt_hi_d/1 -> Cnt_wrap/1  "Cnt_hi_d"
  Cnt_wrap/1 -> Cnt_s/2  "Cnt_wrap"
  State_L/1 -> Fb_L/1  "state"
  State_R/1 -> Fb_R/1  "state"
  Cnt_s/1 -> Cnt_i32/1  "Cnt_s"
  Cnt_i32/1 -> Cnt_dmx/1  "enc_cnt"
  Cnt_dmx/1 -> Fb_L/5  "enc_cnt"
  Cnt_dmx/2 -> Fb_R/5  "enc_cnt"
  Z_u16/1 -> Fb_R/3, Fb_L/3  "fault_code"
  Z_s/1 -> Fb_R/6, Fb_L/6  "tau_est"
  T_peak/1 -> Fb_R/7, Fb_L/7  "tau_avail"
  Z_iq/1 -> Fb_R/8, Fb_L/8  "i_q"
  Z_idc/1 -> Fb_R/9, Fb_L/9  "i_dc"
  Wm_s_L/1 -> Fb_L/4  "w_m"
  Wm_s_R/1 -> Fb_R/4  "w_m"
  V_dc/1 -> Fb_R/10, Fb_L/10  "v_dc"
  T_K/1 -> Fb_R/11, Fb_L/11  "T_motor"
  T_K_esc/1 -> Fb_R/12, Fb_L/12  "T_esc"
  Alive/1 -> Fb_R/14, Fb_L/14  "alive"
  Rx_ok/1 -> Fb_R/15, Fb_L/15  "rx_ok"
  Fb_L/1 -> Pack_L/1  "fb_L"
  Fb_R/1 -> Pack_R/1  "fb_R"
  Node_L/1 -> Pack_L/2  "Node_L"
  Node_R/1 -> Pack_R/2  "Node_R"
  Pack_L/1 -> Drop_fb1_L/1, Drop_fb1_L_sel/1  "Pack_L_1"
  Pack_L/2 -> RT_fb2_L/1  "Pack_L_2"
  Pack_L/3 -> Drop_fb3_L/1, Drop_fb3_L_sel/1  "Pack_L_3"
  Pack_R/1 -> Drop_fb1_R/1, Drop_fb1_R_sel/1  "Pack_R_1"
  Pack_R/2 -> RT_fb2_R/1  "Pack_R_2"
  Pack_R/3 -> Drop_fb3_R/1, Drop_fb3_R_sel/1  "Pack_R_3"
  Drop_fb1_L_sel/1 -> Drop_fb1_L_and/1  "<valid>"
  Drop_fb1_R_sel/1 -> Drop_fb1_R_and/1  "<valid>"
  Drop_fb3_L_sel/1 -> Drop_fb3_L_and/1  "<valid>"
  Drop_fb3_R_sel/1 -> Drop_fb3_R_and/1  "<valid>"
  Drop_fb1_L_and/1 -> Drop_fb1_L/2  "Drop_fb1_L_and"
  Drop_fb1_R_and/1 -> Drop_fb1_R/2  "Drop_fb1_R_and"
  Drop_fb3_L_and/1 -> Drop_fb3_L/2  "Drop_fb3_L_and"
  Drop_fb3_R_and/1 -> Drop_fb3_R/2  "Drop_fb3_R_and"
  RT_fb2_L/1 -> Drop_fb2_L/1, Drop_fb2_L_sel/1  "RT_fb2_L"
  RT_fb2_R/1 -> Drop_fb2_R/1, Drop_fb2_R_sel/1  "RT_fb2_R"
  Drop_fb2_L_sel/1 -> Drop_fb2_L_and/1  "<valid>"
  Drop_fb2_R_sel/1 -> Drop_fb2_R_and/1  "<valid>"
  Drop_fb2_L_and/1 -> Drop_fb2_L/2  "Drop_fb2_L_and"
  Drop_fb2_R_and/1 -> Drop_fb2_R/2  "Drop_fb2_R_and"
  Drop_fb1_L/1 -> Fast_BC/1  "fb1_L"
  Drop_fb1_R/1 -> Fast_BC/2  "fb1_R"
  Drop_fb3_L/1 -> Fast_BC/3  "fb3_L"
  Drop_fb3_R/1 -> Fast_BC/4  "fb3_R"
  Fast_BC/1 -> esc_fast/1  "esc_fast"
  Drop_fb2_L/1 -> Slow_BC/1  "fb2_L"
  Drop_fb2_R/1 -> Slow_BC/2  "fb2_R"
  Slow_BC/1 -> esc_slow/1  "esc_slow"

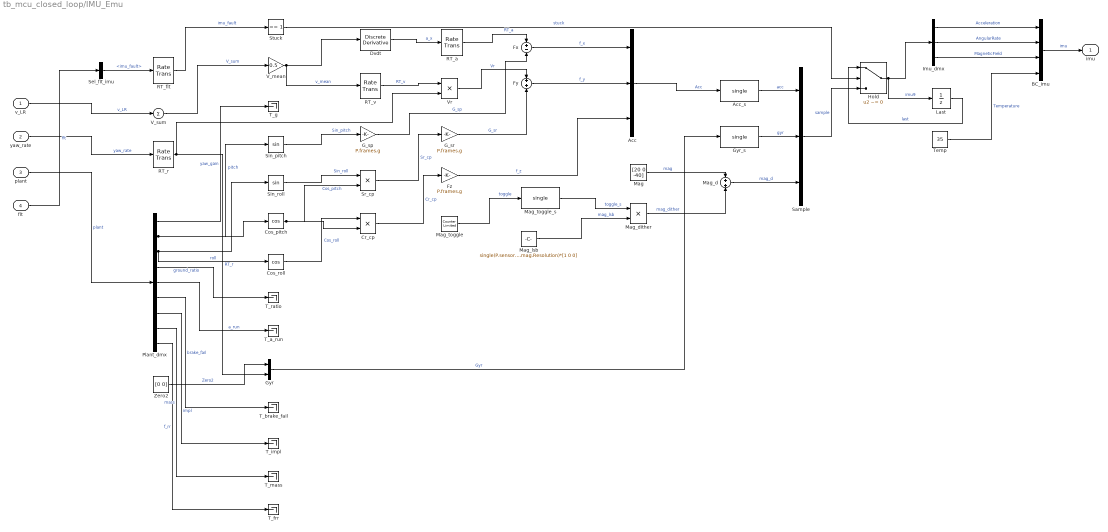
== system tb_mcu_closed_loop/IMU_Emu ==
  v_LR : Inport
  yaw_rate : Inport  Port=2
  plant : Inport  Port=3
  flt : Inport  Port=4
  Acc : Concatenate  NumInputs=3
  Acc_s : DataTypeConversion  OutDataTypeStr=single  RndMeth=Round
  BC_imu : BusCreator  Inputs=4  OutDataTypeStr=Bus: Bus_ImuRaw  NonVirtualBus=on
      settings: InheritFromInputs=off
  Cos_pitch : Trigonometry  Operator=cos
  Cos_roll : Trigonometry  Operator=cos
  Cr_cp : Product  Inputs=**
  Dvdt : simulink/Discrete/Discrete Derivative  gainval=1.0  ICPrevScaledInput=0  OutMin=[]  OutMax=[]  OutDataType=fixdt(1, 16)  OutScaling=2^-10  DoSatur=off
  Fx : Sum  Inputs=+-
  Fy : Sum
  Fz : Gain  Gain=P.frames.g
  G_sp : Gain  Gain=P.frames.g
  G_sr : Gain  Gain=P.frames.g
  Gyr : Concatenate
  Gyr_s : DataTypeConversion  OutDataTypeStr=single  RndMeth=Round
  Hold : Switch  Criteria=u2 ~= 0  SaturateOnIntegerOverflow=off  InputSameDT=off
  Imu_dmx : Demux  Outputs=[3 3 3]
  Last : UnitDelay  SampleTime=Ts.imu
  Mag : Constant  Value=[20 0 -40]  OutDataTypeStr=single  SampleTime=Ts.imu
  Mag_d : Sum
  Mag_dither : Product  Inputs=**
  Mag_lsb : Constant  Value=single(P.sensors.imu.mag.Resolution)*[1 0 0]  OutDataTypeStr=single  SampleTime=Ts.imu
  Mag_toggle : simulink/Sources/Counter Limited  uplimit=1  tsamp=Ts.imu
  Mag_toggle_s : DataTypeConversion  OutDataTypeStr=single  RndMeth=Round
  Plant_dmx : Demux  Outputs=9
  RT_a : RateTransition  OutPortSampleTime=Ts.imu
  RT_flt : RateTransition  OutPortSampleTime=Ts.imu
  RT_r : RateTransition  OutPortSampleTime=Ts.imu
  RT_v : RateTransition  OutPortSampleTime=Ts.imu
  Sample : Concatenate  NumInputs=3
  Sel_flt_imu : BusSelector  OutputSignals=imu_fault
  Sin_pitch : Trigonometry
  Sin_roll : Trigonometry
  Sr_cp : Product  Inputs=**
  Stuck : simulink/Logic and Bit Operations/Compare To Constant  relop===  const=1  OutDataTypeStr=boolean
  T_a_run : Terminator
  T_brake_fail : Terminator
  T_frr : Terminator
  T_g : Terminator
  T_impl : Terminator
  T_mass : Terminator
  T_ratio : Terminator
  Temp : Constant  Value=35  OutDataTypeStr=single  SampleTime=Ts.imu
  V_mean : Gain  Gain=0.5
  V_sum : Sum  Inputs=+
  Vr : Product  Inputs=**
  Zero2 : Constant  Value=[0 0]  OutDataTypeStr=double  SampleTime=Ts.imu
  imu : Outport
  wires:
  v_LR/1 -> V_sum/1  "v_LR"
  yaw_rate/1 -> RT_r/1  "yaw_rate"
  plant/1 -> Plant_dmx/1  "plant"
  flt/1 -> Sel_flt_imu/1  "flt"
  Sel_flt_imu/1 -> RT_flt/1  "<imu_fault>"
  Plant_dmx/1 -> T_g/1  "yaw_gain"
  Plant_dmx/2 -> Sin_pitch/1, Cos_pitch/1  "pitch"
  Plant_dmx/3 -> Sin_roll/1, Cos_roll/1  "roll"
  Plant_dmx/4 -> T_ratio/1  "ground_ratio"
  Plant_dmx/5 -> T_a_run/1  "a_run"
  Plant_dmx/6 -> T_brake_fail/1  "brake_fail"
  Plant_dmx/7 -> T_impl/1  "impl"
  Plant_dmx/8 -> T_mass/1  "mass"
  Plant_dmx/9 -> T_frr/1  "f_rr"
  V_sum/1 -> V_mean/1  "V_sum"
  Zero2/1 -> Gyr/1  "Zero2"
  RT_flt/1 -> Stuck/1  "imu_fault"
  RT_r/1 -> Gyr/2, Vr/2  "RT_r"
  Gyr/1 -> Gyr_s/1  "Gyr"
  Stuck/1 -> Hold/2  "stuck"
  V_mean/1 -> Dvdt/1, RT_v/1  "v_mean"
  Sin_pitch/1 -> G_sp/1  "Sin_pitch"
  Sin_roll/1 -> Sr_cp/1  "Sin_roll"
  Cos_pitch/1 -> Sr_cp/2, Cr_cp/2  "Cos_pitch"
  Cos_roll/1 -> Cr_cp/1  "Cos_roll"
  Sr_cp/1 -> G_sr/1  "Sr_cp"
  Cr_cp/1 -> Fz/1  "Cr_cp"
  RT_v/1 -> Vr/1  "RT_v"
  Dvdt/1 -> RT_a/1  "a_x"
  G_sr/1 -> Fy/2  "G_sr"
  Fz/1 -> Acc/3  "f_z"
  Mag_toggle/1 -> Mag_toggle_s/1  "toggle"
  RT_a/1 -> Fx/1  "RT_a"
  Fx/1 -> Acc/1  "f_x"
  Fy/1 -> Acc/2  "f_y"
  Mag_lsb/1 -> Mag_dither/2  "mag_lsb"
  Mag_toggle_s/1 -> Mag_dither/1  "toggle_s"
  Acc/1 -> Acc_s/1  "Acc"
  Mag/1 -> Mag_d/1  "mag"
  Mag_dither/1 -> Mag_d/2  "mag_dither"
  Mag_d/1 -> Sample/3  "mag_d"
  Acc_s/1 -> Sample/1  "acc"
  Gyr_s/1 -> Sample/2  "gyr"
  Sample/1 -> Hold/3  "sample"
  Hold/1 -> Imu_dmx/1, Last/1  "imu9"
  Imu_dmx/1 -> BC_imu/1  "Acceleration"
  Imu_dmx/2 -> BC_imu/2  "AngularRate"
  Imu_dmx/3 -> BC_imu/3  "MagneticField"
  Temp/1 -> BC_imu/4  "Temperature"
  Last/1 -> Hold/1  "last"
  BC_imu/1 -> imu/1  "imu"
  G_sp/1 -> Fx/2  "G_sp"
  Vr/1 -> Fy/1  "Vr"

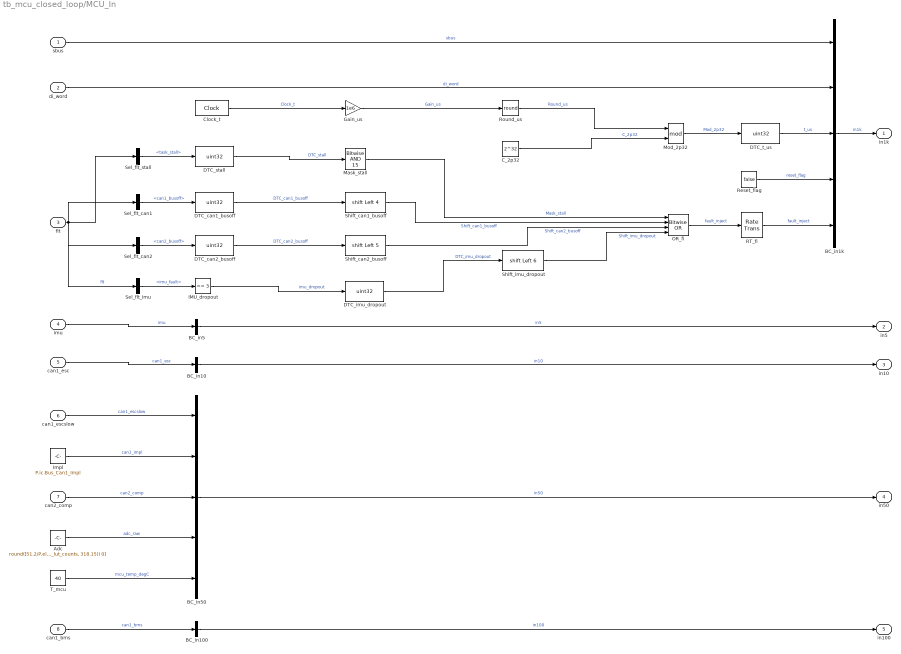
== system tb_mcu_closed_loop/MCU_In ==
  sbus : Inport
  di_word : Inport  Port=2
  flt : Inport  Port=3
  imu : Inport  Port=4
  can1_esc : Inport  Port=5
  can1_escslow : Inport  Port=6
  can2_comp : Inport  Port=7
  can1_bms : Inport  Port=8
  Adc : Constant  Value=round([51.2/P.electronics.adc.k_vpack 51.2/P.electronics.adc.k_vlink P.electronics.adc.i_off 24/P.electronics.adc.k_v24 12/P.electronics.adc.k_v12 5/P.electronics.adc.k_v5 0 0.5*P.electronics.adc.vref]/P.electronics.adc.vref*65535) + [0 0 0 0 0 0 round(interp1(P.electronics.adc.ntc_lut_K, P.electronics.adc.ntc_lut_counts, 318.15)) 0]  OutDataTypeStr=uint16  SampleTime=Ts.comm
  BC_in10 : BusCreator  Inputs=1  OutDataTypeStr=Bus: Bus_McuIn10  NonVirtualBus=on
      settings: InheritFromInputs=off
  BC_in100 : BusCreator  Inputs=1  OutDataTypeStr=Bus: Bus_McuIn100  NonVirtualBus=on
      settings: InheritFromInputs=off
  BC_in1k : BusCreator  Inputs=5  OutDataTypeStr=Bus: Bus_McuIn1k  NonVirtualBus=on
      settings: InheritFromInputs=off
  BC_in5 : BusCreator  Inputs=1  OutDataTypeStr=Bus: Bus_McuIn5  NonVirtualBus=on
      settings: InheritFromInputs=off
  BC_in50 : BusCreator  Inputs=5  OutDataTypeStr=Bus: Bus_McuIn50  NonVirtualBus=on
      settings: InheritFromInputs=off
  C_2p32 : Constant  Value=2^32  OutDataTypeStr=double  SampleTime=Ts.base
  Clock_t : DigitalClock  SampleTime=Ts.base
  DTC_can1_busoff : DataTypeConversion  OutDataTypeStr=uint32  RndMeth=Round
  DTC_can2_busoff : DataTypeConversion  OutDataTypeStr=uint32  RndMeth=Round
  DTC_imu_dropout : DataTypeConversion  OutDataTypeStr=uint32  RndMeth=Round
  DTC_stall : DataTypeConversion  OutDataTypeStr=uint32  RndMeth=Round
  DTC_t_us : DataTypeConversion  OutDataTypeStr=uint32  SaturateOnIntegerOverflow=off  RndMeth=Floor
  Gain_us : Gain  Gain=1e6
  IMU_dropout : simulink/Logic and Bit Operations/Compare To Constant  relop===  const=3  OutDataTypeStr=boolean
  Impl : Constant  Value=P.ic.Bus_Can1_Impl  OutDataTypeStr=Bus: Bus_Can1_Impl  SampleTime=Ts.comm
  Mask_stall : simulink/Logic and Bit Operations/Bitwise Operator  logicop=AND  UseBitMask=on  BitMask=15  BitMaskRealWorld=Stored Integer
  Mod_2p32 : Math  Operator=mod
  OR_fi : simulink/Logic and Bit Operations/Bitwise Operator  logicop=OR  UseBitMask=off  NumInputPorts=4  BitMask=bin2dec('11011001')  BitMaskRealWorld=Stored Integer
  RT_fi : RateTransition  OutPortSampleTime=Ts.base
  Reset_flag : Constant  Value=false  OutDataTypeStr=boolean  SampleTime=Ts.base
  Round_us : Rounding  Operator=round
  Sel_flt_can1 : BusSelector  OutputSignals=can1_busoff
  Sel_flt_can2 : BusSelector  OutputSignals=can2_busoff
  Sel_flt_imu : BusSelector  OutputSignals=imu_fault
  Sel_flt_stall : BusSelector  OutputSignals=task_stall
  Shift_can1_busoff : ArithShift  BitShiftNumber=4  BitShiftDirection=Left
  Shift_can2_busoff : ArithShift  BitShiftNumber=5  BitShiftDirection=Left
  Shift_imu_dropout : ArithShift  BitShiftNumber=6  BitShiftDirection=Left
  T_mcu : Constant  Value=40  OutDataTypeStr=single  SampleTime=Ts.comm
  in1k : Outport
  in5 : Outport  Port=2
  in10 : Outport  Port=3
  in50 : Outport  Port=4
  in100 : Outport  Port=5
  wires:
  sbus/1 -> BC_in1k/1  "sbus"
  di_word/1 -> BC_in1k/2  "di_word"
  flt/1 -> Sel_flt_stall/1, Sel_flt_imu/1, Sel_flt_can2/1, Sel_flt_can1/1  "flt"
  imu/1 -> BC_in5/1  "imu"
  can1_esc/1 -> BC_in10/1  "can1_esc"
  can1_escslow/1 -> BC_in50/1  "can1_escslow"
  Impl/1 -> BC_in50/2  "can1_impl"
  can2_comp/1 -> BC_in50/3  "can2_comp"
  Adc/1 -> BC_in50/4  "adc_raw"
  T_mcu/1 -> BC_in50/5  "mcu_temp_degC"
  can1_bms/1 -> BC_in100/1  "can1_bms"
  Sel_flt_stall/1 -> DTC_stall/1  "<task_stall>"
  Sel_flt_can1/1 -> DTC_can1_busoff/1  "<can1_busoff>"
  Sel_flt_can2/1 -> DTC_can2_busoff/1  "<can2_busoff>"
  Sel_flt_imu/1 -> IMU_dropout/1  "<imu_fault>"
  BC_in5/1 -> in5/1  "in5"
  BC_in10/1 -> in10/1  "in10"
  BC_in50/1 -> in50/1  "in50"
  BC_in100/1 -> in100/1  "in100"
  IMU_dropout/1 -> DTC_imu_dropout/1  "imu_dropout"
  Clock_t/1 -> Gain_us/1  "Clock_t"
  DTC_stall/1 -> Mask_stall/1  "DTC_stall"
  DTC_can1_busoff/1 -> Shift_can1_busoff/1  "DTC_can1_busoff"
  DTC_can2_busoff/1 -> Shift_can2_busoff/1  "DTC_can2_busoff"
  Gain_us/1 -> Round_us/1  "Gain_us"
  Mask_stall/1 -> OR_fi/1  "Mask_stall"
  DTC_imu_dropout/1 -> Shift_imu_dropout/1  "DTC_imu_dropout"
  Shift_can1_busoff/1 -> OR_fi/2  "Shift_can1_busoff"
  Shift_can2_busoff/1 -> OR_fi/3  "Shift_can2_busoff"
  Round_us/1 -> Mod_2p32/1  "Round_us"
  C_2p32/1 -> Mod_2p32/2  "C_2p32"
  Shift_imu_dropout/1 -> OR_fi/4  "Shift_imu_dropout"
  Mod_2p32/1 -> DTC_t_us/1  "Mod_2p32"
  OR_fi/1 -> RT_fi/1  "fault_inject"
  Reset_flag/1 -> BC_in1k/4  "reset_flag"
  RT_fi/1 -> BC_in1k/5  "fault_inject"
  DTC_t_us/1 -> BC_in1k/3  "t_us"
  BC_in1k/1 -> in1k/1  "in1k"

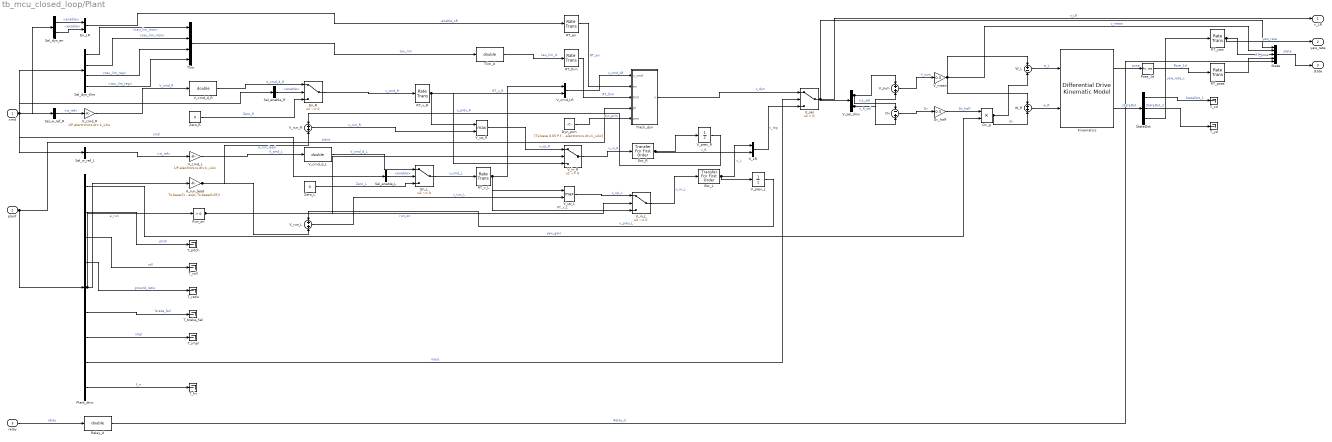
== system tb_mcu_closed_loop/Plant ==
  cmd : Inport
  plant : Inport  Port=2
  relay : Inport  Port=3
  A_run_lead : Gain  Gain=Ts.base/(1 - exp(-Ts.base/0.05))
  Dv : Sum  Inputs=-+
  Dv_g : Product  Inputs=**
  Dv_half : Gain  Gain=0.5
  Dyn_prm : Constant  Value=[Ts.base 0.05 P.frames.g P.electronics.drv.k_v2w]  OutDataTypeStr=double  SampleTime=Ts.base
  En_L : Switch  Criteria=u2 ~= 0  SaturateOnIntegerOverflow=off  InputSameDT=off
  En_LR : Concatenate
  En_R : Switch  Criteria=u2 ~= 0  SaturateOnIntegerOverflow=off  InputSameDT=off
  Esc_L : simulink/Discrete/Transfer Fcn First Order  PoleZ=exp(-Ts.base/0.05)  ICPrevOutput=0  DoSatur=off
  Esc_R : simulink/Discrete/Transfer Fcn First Order  PoleZ=exp(-Ts.base/0.05)  ICPrevOutput=0  DoSatur=off
  Kinematics : robotmobilelib/Differential Drive Kinematic Model  VehicleInputs=Wheel Speeds  WheelRadius=1  WheelSpeedRange=[-inf inf]  TrackWidth=P.electronics.mix.chi*P.electronics.mix.B  InitialState=[0; 0; 0]  SimulateUsing=Code generation
  Plant_dmx : Demux  Outputs=9
  Pose_1d : Reshape
  RT_en : RateTransition  InitialCondition=false  OutPortSampleTime=Ts.base
  RT_pose : RateTransition  InitialCondition=[0 0 0]  OutPortSampleTime=Ts.base
  RT_tlim : RateTransition  InitialCondition=[0 0 0 0]  OutPortSampleTime=Ts.base
  RT_v_L : RateTransition  OutPortSampleTime=Ts.base
  RT_v_R : RateTransition  OutPortSampleTime=Ts.base
  RT_yaw : RateTransition  OutPortSampleTime=Ts.base
  Relay_d : DataTypeConversion  OutDataTypeStr=double  RndMeth=Round
  Run_on : simulink/Logic and Bit Operations/Compare To Zero  relop=>  OutDataTypeStr=boolean
  Sel_dyn_en : BusSelector  OutputSignals=L.enable,R.enable
  Sel_dyn_tlim : BusSelector  OutputSignals=L.tau_lim_mot,R.tau_lim_mot,L.tau_lim_reg,R.tau_lim_reg
  Sel_enable_L : BusSelector  OutputSignals=L.enable
  Sel_enable_R : BusSelector  OutputSignals=R.enable
  Sel_w_ref_L : BusSelector  OutputSignals=L.w_ref
  Sel_w_ref_R : BusSelector  OutputSignals=R.w_ref
  State : Concatenate  NumInputs=5
  StateDot : Demux  Outputs=3
  T_brake_fail : Terminator
  T_frr : Terminator
  T_impl : Terminator
  T_pitch : Terminator
  T_ratio : Terminator
  T_roll : Terminator
  T_xd : Terminator
  T_yd : Terminator
  Tlim : Concatenate  NumInputs=4
  Tlim_d : DataTypeConversion  OutDataTypeStr=double  RndMeth=Round
  Track_dyn : MATLAB Function  TreatAsAtomicUnit=on
  V_LR : Concatenate
  V_cmd_L : Gain  Gain=1/P.electronics.drv.k_v2w
  V_cmd_LR : Concatenate
  V_cmd_R : Gain  Gain=1/P.electronics.drv.k_v2w
  V_cmd_d_L : DataTypeConversion  OutDataTypeStr=double  RndMeth=Round
  V_cmd_d_R : DataTypeConversion  OutDataTypeStr=double  RndMeth=Round
  V_in_L : Switch  Criteria=u2 ~= 0  SaturateOnIntegerOverflow=off  InputSameDT=off
  V_in_R : Switch  Criteria=u2 ~= 0  SaturateOnIntegerOverflow=off  InputSameDT=off
  V_mean : Gain  Gain=0.5
  V_prev_L : UnitDelay  SampleTime=Ts.base
  V_prev_R : UnitDelay  SampleTime=Ts.base
  V_run_L : Sum
  V_run_R : Sum
  V_sel : Switch  Criteria=u2 > Threshold  SaturateOnIntegerOverflow=off  InputSameDT=off
  V_sel_dmx : Demux  Outputs=2
  V_sum : Sum
  V_up_L : MinMax  Function=max  Inputs=2
  V_up_R : MinMax  Function=max  Inputs=2
  W_L : Sum  Inputs=+-
  W_R : Sum
  Zero_L : Constant  Value=0  OutDataTypeStr=double  SampleTime=Ts.ctrl
  Zero_R : Constant  Value=0  OutDataTypeStr=double  SampleTime=Ts.ctrl
  v_LR : Outport
  yaw_rate : Outport  Port=2
  state : Outport  Port=3
  wires:
  cmd/1 -> Sel_dyn_en/1, Sel_enable_L/1, Sel_dyn_tlim/1, Sel_w_ref_L/1, Sel_enable_R/1, Sel_w_ref_R/1  "cmd"
  plant/1 -> Track_dyn/4(pl), Plant_dmx/1  "plant"
  relay/1 -> Relay_d/1  "relay"
  Sel_dyn_en/1 -> En_LR/1  "<enable>"
  Sel_dyn_en/2 -> En_LR/2  "<enable>"
  Sel_w_ref_R/1 -> V_cmd_R/1  "<w_ref>"
  En_LR/1 -> RT_en/1  "enable_LR"
  Sel_dyn_tlim/1 -> Tlim/1  "<tau_lim_mot>"
  Sel_dyn_tlim/2 -> Tlim/2  "<tau_lim_mot>"
  Sel_dyn_tlim/3 -> Tlim/3  "<tau_lim_reg>"
  Sel_dyn_tlim/4 -> Tlim/4  "<tau_lim_reg>"
  Sel_w_ref_L/1 -> V_cmd_L/1  "<w_ref>"
  Plant_dmx/1 -> Dv_g/2  "yaw_gain"
  Plant_dmx/2 -> T_pitch/1  "pitch"
  Plant_dmx/3 -> T_roll/1  "roll"
  Plant_dmx/4 -> T_ratio/1  "ground_ratio"
  Plant_dmx/5 -> A_run_lead/1, Run_on/1  "a_run"
  Plant_dmx/6 -> T_brake_fail/1  "brake_fail"
  Plant_dmx/7 -> T_impl/1  "impl"
  Plant_dmx/8 -> V_sel/2  "mass"
  Plant_dmx/9 -> T_frr/1  "f_rr"
  V_cmd_R/1 -> V_cmd_d_R/1  "V_cmd_R"
  Relay_d/1 -> State/5  "Relay_d"
  Tlim/1 -> Tlim_d/1  "tau_lim"
  Zero_R/1 -> En_R/3  "Zero_R"
  V_cmd_L/1 -> V_cmd_d_L/1  "V_cmd_L"
  A_run_lead/1 -> V_run_R/2, V_run_L/2  "a_run_lead"
  Run_on/1 -> V_in_R/2, V_in_L/2  "run_on"
  V_cmd_d_R/1 -> En_R/1  "V_cmd_d_R"
  Sel_enable_R/1 -> En_R/2  "<enable>"
  V_run_R/1 -> V_up_R/2  "v_run_R"
  V_run_L/1 -> V_up_L/2  "v_run_L"
  Zero_L/1 -> En_L/3  "Zero_L"
  En_R/1 -> RT_v_R/1  "v_cmd_R"
  V_cmd_d_L/1 -> En_L/1  "V_cmd_d_L"
  Sel_enable_L/1 -> En_L/2  "<enable>"
  RT_v_R/1 -> V_in_R/3, V_up_R/1, V_cmd_LR/2  "RT_v_R"
  En_L/1 -> RT_v_L/1  "v_cmd_L"
  V_up_R/1 -> V_in_R/1  "v_up_R"
  RT_v_L/1 -> V_cmd_LR/1, V_in_L/3, V_up_L/1  "RT_v_L"
  Tlim_d/1 -> RT_tlim/1  "tau_lim_d"
  V_cmd_LR/1 -> Track_dyn/1(v_cmd)  "v_cmd_LR"
  Dyn_prm/1 -> Track_dyn/5(prm)  "dyn_prm"
  V_up_L/1 -> V_in_L/1  "v_up_L"
  RT_en/1 -> Track_dyn/2(en)  "RT_en"
  RT_tlim/1 -> Track_dyn/3(tlim)  "RT_tlim"
  V_in_R/1 -> Esc_R/1  "v_in_R"
  V_in_L/1 -> Esc_L/1  "v_in_L"
  Esc_R/1 -> V_prev_R/1, V_LR/2  "v_R"
  Track_dyn/1(v) -> V_sel/1  "v_dyn"
  V_prev_R/1 -> V_run_R/1  "v_prev_R"
  Esc_L/1 -> V_LR/1, V_prev_L/1  "v_L"
  V_LR/1 -> V_sel/3  "v_lag"
  V_prev_L/1 -> V_run_L/1  "v_prev_L"
  V_sel/1 -> v_LR/1, State/1, V_sel_dmx/1  "v_LR"
  V_sel_dmx/1 -> V_sum/1, Dv/1  "v_L_sel"
  V_sel_dmx/2 -> V_sum/2, Dv/2  "v_R_sel"
  V_sum/1 -> V_mean/1  "V_sum"
  Dv/1 -> Dv_half/1  "Dv"
  Dv_half/1 -> Dv_g/1  "Dv_half"
  W_L/1 -> Kinematics/1  "w_L"
  W_R/1 -> Kinematics/2  "w_R"
  Kinematics/1 -> Pose_1d/1  "pose"
  Kinematics/2 -> StateDot/1  "stateDot"
  StateDot/1 -> T_xd/1  "StateDot_1"
  StateDot/2 -> T_yd/1  "StateDot_2"
  StateDot/3 -> RT_yaw/1  "yaw_rate_c"
  Pose_1d/1 -> RT_pose/1  "Pose_1d"
  RT_yaw/1 -> State/3, yaw_rate/1  "yaw_rate"
  RT_pose/1 -> State/4  "RT_pose"
  State/1 -> state/1  "state"
  V_mean/1 -> State/2, W_R/1, W_L/1  "v_mean"
  Dv_g/1 -> W_L/2, W_R/2  "dv"
